simulink model "LineFollower_P_Controller"  (R2024b)
settings: Solver=FixedStepDiscrete  StartTime=0.0  StopTime=inf  FixedStep=0.01  RelTol=1e-3
settings Model: Creator=Devansh  LastModifiedBy=Devansh

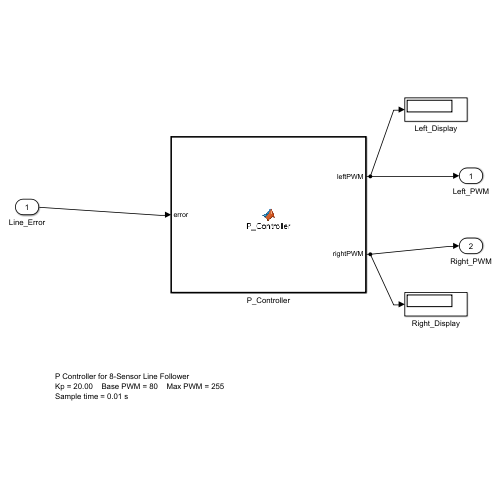
[thumbnail: Simulink's stored preview of the top-level diagram]
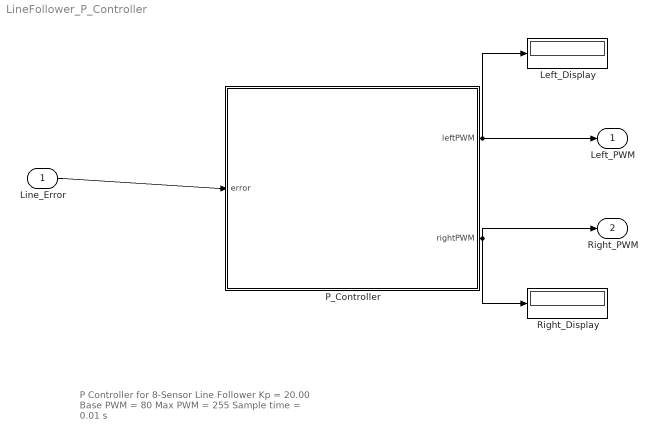
== system LineFollower_P_Controller ==
  note: P Controller for 8-Sensor Line Follower
      | Kp = 20.00    Base PWM = 80    Max PWM = 255
      | Sample time = 0.01 s
  Line_Error : Inport
  Left_Display : Display
  P_Controller : MATLAB Function  TreatAsAtomicUnit=on
  Right_Display : Display
  Left_PWM : Outport
  Right_PWM : Outport  Port=2
  wires:
  Line_Error/1 -> P_Controller/1(error)
  P_Controller/1(leftPWM) -> Left_Display/1, Left_PWM/1
  P_Controller/2(rightPWM) -> Right_Display/1, Right_PWM/1

== matlab function LineFollower_P_Controller/P_Controller ==
  data: error input; leftPWM output; rightPWM output
function [leftPWM,rightPWM] = P_Controller(error)
%#codegen

Kp = 20.00;
basePWM = 80.00;
maxPWM = 255.00;

correction = Kp * error;

leftPWM = basePWM + correction;
rightPWM = basePWM - correction;

if leftPWM > maxPWM
    leftPWM = maxPWM;
end

if leftPWM < 0
    leftPWM = 0;
end

if rightPWM > maxPWM
    rightPWM = maxPWM;
end

if rightPWM < 0
    rightPWM = 0;
end

end
